simulink model "MIMO_code_pll_v2_r2016b"  (R2016b)
settings: Solver=FixedStepDiscrete  StartTime=0.0  StopTime=30  FixedStep=Ts  RelTol=1e-3
InitFcn:
  | Ts = 50e-6;
libraries: powerlib x16, powerlib_meascontrol x4
settings Model: Creator=ym  LastModifiedBy=ncepri14

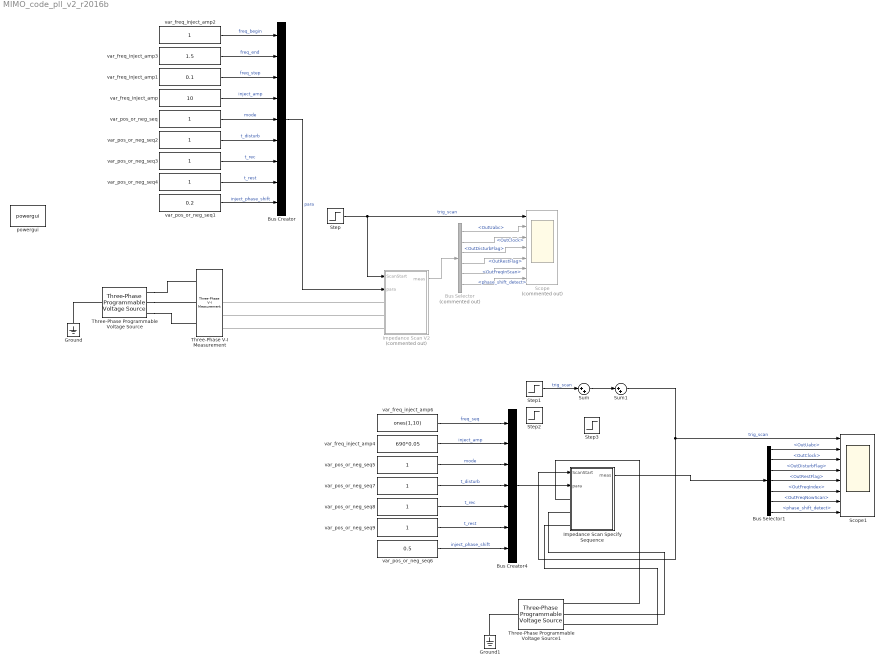
== system MIMO_code_pll_v2_r2016b ==
  Bus Creator : BusCreator  Inputs=9
  Bus Creator4 : BusCreator  Inputs=7
  Bus Selector : BusSelector  Commented=on  OutputSignals=scan_module_meas.OutUabc,scan_module_meas.OutClock,scan_module_meas.OutDisturbFlag,scan_module_meas.OutRestFlag,scan_module_meas.OutFreqInScan,phase_shift_detect
  Bus Selector1 : BusSelector  OutputSignals=scan_module_meas.OutUabc,scan_module_meas.OutClock,scan_module_meas.OutDisturbFlag,scan_module_meas.OutRestFlag,scan_module_meas.OutFreqIndex,scan_module_meas.OutFreqNowScan,phase_shift_detect
  Ground : powerlib/Elements/Ground  LConnTagsString=a
  Ground1 : powerlib/Elements/Ground  LConnTagsString=a
  Impedance Scan Specify Sequence : Subsystem  mask{var_gui_external=External, var_t_start=2, var_freq_seq=[1:350], var_inject_duration=1, var_record_duration=1, var_rest_duration=2, var_inject_amp=690*0.05, var_inject_mode=1, var_inject_phase_shift=0, var_ts=50e-6}
      mask prompts: var_gui_external "Using"; var_t_start "Injection starting time (s)"; var_freq_seq "Frequency Sequence (Hz)"; var_inject_duration "Injection durtion (s)"; var_record_duration "Record duration (s), this set only output a recording signal"; var_rest_duration "Stable durtion (s)"; var_inject_amp "Injection magnitude. eg. 690*0.02"; var_inject_mode "Injection mode. eg 1 for Positive sequence, 2 for Negative, 3 for MIMO"; var_inject_phase_shift "Injection phase shift angle (deg). eg. if set 20 deg, disturb will injected when the phase angle 20deg of grid Uabc comes"; var_ts "Sample time"
      mask help:
      | |--------------Injection duration--------------|-----Stable duration------|
      |                      |-----Record duration-----|
      |
      | Record duration <= Inject duration
      |
      | Freq coupling implemented in this version
      mask init:
      | block = find_system(gcb,...
      |           'LookUnderMasks','on',...
      |           'FollowLinks','on','Name','In2');
      | % p=Simulink.Mask.get(gcb);
      | 
      | maskObj = Simulink.Mask.get(gcb);
      | [control, phandle] = maskObj.getDialogControl('para_group_gui_setting_zone');
      | 
      | switch var_gui_external
      |     case 1
      |         
      | %       if ~isempty(block)
      | % %         delete_block(block);
      | %         
      | %       end
      |       control.Visible = 'on';
      | 
      |       
      |       
      | %       p.getDialogControl('para_group_gui_setting_zone').Visible='on';
      |     case 2
      |         
      | %         if isempty(block)
      | % %             add_block('built-in/Inport',[gcb,'/In2']);
      | %         end
      |         
      |         control.Visible = 'off';
      | %         p.getDialogControl('para_group_gui_setting_zone').Visible='off';
      | end % switch
      | 
      | disp(num2str(var_gui_external));
      mask Help:
      | by Yamin
      | v2(2024/5/17):
      | 1. add PLL phase alignment;
      | 2. Frequence sequence now can be specified by vector, elements could be random if you intend to do so.
      mask TypeOptions var_gui_external: GUI | External
  Impedance Scan V2 : Subsystem  Commented=on  mask{var_gui_external=External, t_start=2, freq_begin=1, freq_end=10, freq_step=1, inject_duration=1, record_duration=1, stable_duration=2, amp_inject=1, inject_mode=1, inject_phase_shift=30, var_ts=50e-6}
      mask prompts: var_gui_external "Using"; t_start "Injection starting time (s)"; freq_begin "Frequency begin (Hz)"; freq_end "Frequncy end (Hz)"; freq_step "Frequency step (Hz)"; inject_duration "Injection durtion (s)"; record_duration "Record duration (s), this set only output a recording signal"; stable_duration "Stable durtion (s)"; amp_inject "Injection magnitude. eg. 690*0.02"; inject_mode "Injection mode. eg 1 for Positive sequence, 2 for Negative, 3 for MIMO"; inject_phase_shift "Injection phase shift angle (deg). eg. if set 20 deg, disturb will injected when the phase angle 20deg of grid Uabc comes"; var_ts "Sample time"
      mask help:
      | |--------------Injection duration--------------|-----Stable duration------|
      |                      |-----Record duration-----|
      |
      | Record duration <= Inject duration
      |
      | Freq coupling implemented in this version
      mask init: same as MIMO_code_pll_v2_r2016b/Impedance Scan Specify Sequence
      mask Help: by Yamin
      mask TypeOptions var_gui_external: GUI | External
  Scope : Scope  Commented=on  NumInputPorts=7
  Scope1 : Scope  NumInputPorts=8
  Step : Step  SampleTime=0
  Step1 : Step  SampleTime=0
  Step2 : Step  Time=2  After=-1  SampleTime=0
  Step3 : Step  Time=5  SampleTime=0
  Sum : Sum  Inputs=|++
  Sum1 : Sum  Inputs=|++
  Three-Phase Programmable Voltage Source : powerlib/Electrical Sources/Three-Phase Programmable Voltage Source  PositiveSequence="[100  0 60]"  VariationEntity=None  VariationType=Table of time-amplitude pairs  VariationTypeAlt=Step  VariationStep=0.5  VariationRate=10  VariationMagnitude=0.3  VariationFrequency=2  VariationTiming=[1 2]  VariationPhaseA=off  Amplitudes=[1 0.8 1.2 1.0]  TimeValues=[0 0.1 0.15 0.2]  HarmonicGeneration=off  HarmonicA=[3 0.2 -25 0]  HarmonicB=[2 0.15 35 2]  Timing="[0.05  3]"  BusType=swing  Pref=0  Qref=0  Qmin=-inf  Qmax=inf
  Three-Phase Programmable Voltage Source1 : powerlib/Electrical Sources/Three-Phase Programmable Voltage Source  PositiveSequence="[100  0 60]"  VariationEntity=None  VariationType=Table of time-amplitude pairs  VariationTypeAlt=Step  VariationStep=0.5  VariationRate=10  VariationMagnitude=0.3  VariationFrequency=2  VariationTiming=[1 2]  VariationPhaseA=off  Amplitudes=[1 0.8 1.2 1.0]  TimeValues=[0 0.1 0.15 0.2]  HarmonicGeneration=off  HarmonicA=[3 0.2 -25 0]  HarmonicB=[2 0.15 35 2]  Timing="[0.05  3]"  BusType=swing  Pref=0  Qref=0  Qmin=-inf  Qmax=inf
  Three-Phase V-I Measurement : powerlib/Measurements/Three-Phase V-I Measurement  VoltageMeasurement=phase-to-ground  SetLabelV=off  LabelV=Vabc  Vpu=off  VpuLL=off  CurrentMeasurement=yes  SetLabelI=off  LabelI=Iabc  Ipu=off  Pbase=100e6  Vbase=500e3  OutputType=Complex  PhasorSimulation=off  PSBequivalent=0
  powergui : powerlib/powergui  Priority=1  SimulationMode=Discrete  SolverType=Tustin/Backward Euler (TBE)  SampleTime=Ts  frequency=60  SPID=off  DisableSnubberDevices=off  DisableRonSwitches=off  DisableVfSwitches=off  SwTol=0  DisplayEquations=off  Interpol=off  ExternalGateDelay=off  methode=off  Ts=10  FunctionMessages=off  echomessages=off  HookPort=off  EnableUseOfTLC=off  x0status=blocks  frequencyindice=60  Pbase=100e6  ErrMax=1e-4  Iterations=50  UnitsV=kV  UnitsW=MW  buscounter=0  RestoreLinks=warning  ResistiveCurrentMeasurement=off  Frange=[0:2:500]  Ylog=off  Xlog=on  ShowGrid=off  save=off  variable=ZData  structure=0  ZoomFFT=off  StartTime=0.0  cycles=1  DisplayStyle=1  fundamental=60  FreqAxis=off  MaxFrequency=1000  frequencyindicesteady=1  RmsSteady=1  display=off
  var_freq_inject_amp : Constant  Value=10
  var_freq_inject_amp1 : Constant  Value=0.1
  var_freq_inject_amp2 : Constant
  var_freq_inject_amp3 : Constant  Value=1.5
  var_freq_inject_amp4 : Constant  Value=690*0.05
  var_freq_inject_amp6 : Constant  Value=ones(1,10)
  var_pos_or_neg_seq{,2..5,7..9} (8 alike) : Constant
  var_pos_or_neg_seq1 : Constant  Value=0.2
  var_pos_or_neg_seq6 : Constant  Value=0.5
  wires:
  Impedance Scan V2/1(meas) -> Bus Selector/1
  var_freq_inject_amp1/1 -> Bus Creator/3  "freq_step"
  var_freq_inject_amp/1 -> Bus Creator/4  "inject_amp"
  var_pos_or_neg_seq/1 -> Bus Creator/5  "mode"
  var_pos_or_neg_seq2/1 -> Bus Creator/6  "t_disturb"
  var_pos_or_neg_seq3/1 -> Bus Creator/7  "t_rec"
  var_pos_or_neg_seq4/1 -> Bus Creator/8  "t_rest"
  var_freq_inject_amp2/1 -> Bus Creator/1  "freq_begin"
  var_freq_inject_amp3/1 -> Bus Creator/2  "freq_end"
  Step/1 -> Impedance Scan V2/1(ScanStart), Scope/1  "trig_scan"
  Bus Creator/1 -> Impedance Scan V2/2(para)  "para"
  var_pos_or_neg_seq1/1 -> Bus Creator/9  "inject_phase_shift"
  Bus Selector/3 -> Scope/4  "<OutDisturbFlag>"
  Bus Selector/2 -> Scope/3  "<OutClock>"
  Bus Selector/4 -> Scope/5  "<OutRestFlag>"
  Bus Selector/1 -> Scope/2  "<OutUabc>"
  Bus Selector/5 -> Scope/6  "<OutFreqInScan>"
  Bus Selector/6 -> Scope/7  "<phase_shift_detect>"
  var_freq_inject_amp4/1 -> Bus Creator4/2  "inject_amp"
  var_pos_or_neg_seq5/1 -> Bus Creator4/3  "mode"
  var_pos_or_neg_seq7/1 -> Bus Creator4/4  "t_disturb"
  var_pos_or_neg_seq8/1 -> Bus Creator4/5  "t_rec"
  var_pos_or_neg_seq9/1 -> Bus Creator4/6  "t_rest"
  var_freq_inject_amp6/1 -> Bus Creator4/1  "freq_seq"
  var_pos_or_neg_seq6/1 -> Bus Creator4/7  "inject_phase_shift"
  Bus Creator4/1 -> Impedance Scan Specify Sequence/2(para)
  Impedance Scan Specify Sequence/1(meas) -> Bus Selector1/1
  Sum1/1 -> Impedance Scan Specify Sequence/1(ScanStart), Scope1/1  "trig_scan"
  Step1/1 -> Sum/1  "trig_scan"
  Sum/1 -> Sum1/1
  Bus Selector1/4 -> Scope1/5  "<OutRestFlag>"
  Bus Selector1/3 -> Scope1/4  "<OutDisturbFlag>"
  Bus Selector1/5 -> Scope1/6  "<OutFreqIndex>"
  Bus Selector1/2 -> Scope1/3  "<OutClock>"
  Bus Selector1/6 -> Scope1/7  "<OutFreqNowScan>"
  Bus Selector1/1 -> Scope1/2  "<OutUabc>"
  Bus Selector1/7 -> Scope1/8  "<phase_shift_detect>"
  connections:
  Three-Phase Programmable Voltage Source/RConn3 -- Three-Phase V-I Measurement/LConn3
  Three-Phase Programmable Voltage Source/RConn2 -- Three-Phase V-I Measurement/LConn2
  Three-Phase Programmable Voltage Source/RConn1 -- Three-Phase V-I Measurement/LConn1
  Impedance Scan V2/LConn3 -- Three-Phase V-I Measurement/RConn3
  Impedance Scan V2/LConn2 -- Three-Phase V-I Measurement/RConn2
  Impedance Scan V2/LConn1 -- Three-Phase V-I Measurement/RConn1
  Ground/LConn1 -- Three-Phase Programmable Voltage Source/LConn1
  Ground1/LConn1 -- Three-Phase Programmable Voltage Source1/LConn1
  Impedance Scan Specify Sequence/LConn1 -- Three-Phase Programmable Voltage Source1/RConn1
  Impedance Scan Specify Sequence/LConn3 -- Three-Phase Programmable Voltage Source1/RConn3
  Impedance Scan Specify Sequence/LConn2 -- Three-Phase Programmable Voltage Source1/RConn2

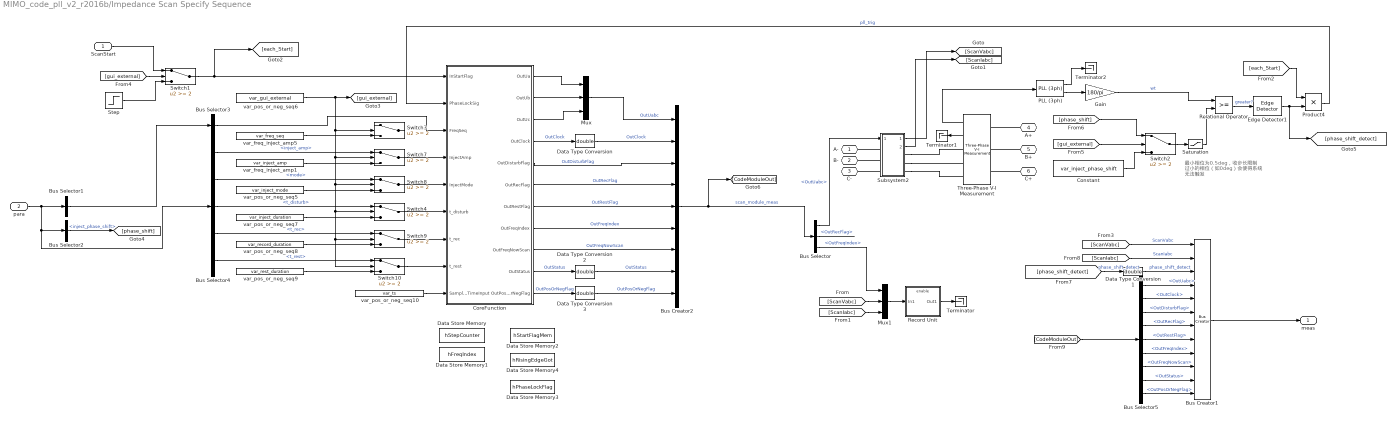
== system MIMO_code_pll_v2_r2016b/Impedance Scan Specify Sequence ==
  note: 最小相位为0.5deg，收步长限制
      | 过小的相位（如0deg）会使得系统
      | 无法触发
  ScanStart : Inport
  para : Inport  Port=2
  Bus Creator1 : BusCreator  Inputs=12
  Bus Creator2 : BusCreator  Inputs=9
  Bus Selector : BusSelector  OutputSignals=OutUabc,OutRecFlag,OutFreqIndex
  Bus Selector1 : BusSelector  OutputSignals=freq_seq,inject_amp,mode,t_disturb,t_rec,t_rest  OutputAsBus=on
  Bus Selector2 : BusSelector  OutputSignals=inject_phase_shift
  Bus Selector3 : BusSelector  OutputSignals=freq_seq  OutputAsBus=on
  Bus Selector4 : BusSelector  OutputSignals=inject_amp,mode,t_disturb,t_rec,t_rest
  Bus Selector5 : BusSelector  OutputSignals=OutUabc,OutClock,OutDisturbFlag,OutRecFlag,OutRestFlag,OutFreqIndex,OutFreqNowScan,OutStatus,OutPosOrNegFlag
  Constant : Constant  Value=var_inject_phase_shift
  CoreFunction : MATLAB Function  TreatAsAtomicUnit=on  SystemSampleTime=var_ts
  Data Store Memory : DataStoreMemory  DataStoreName=hStepCounter  ReadBeforeWriteMsg=warning  WriteAfterWriteMsg=warning  WriteAfterReadMsg=warning  ShowAdditionalParam=off  OutDataTypeStr=int32
  Data Store Memory1 : DataStoreMemory  DataStoreName=hFreqIndex  ReadBeforeWriteMsg=warning  WriteAfterWriteMsg=warning  WriteAfterReadMsg=warning  ShowAdditionalParam=off  OutDataTypeStr=double
  Data Store Memory2 : DataStoreMemory  DataStoreName=hStartFlagMem  ReadBeforeWriteMsg=warning  WriteAfterWriteMsg=warning  WriteAfterReadMsg=warning  ShowAdditionalParam=off  OutDataTypeStr=int32
  Data Store Memory3 : DataStoreMemory  DataStoreName=hPhaseLockFlag  ReadBeforeWriteMsg=warning  WriteAfterWriteMsg=warning  WriteAfterReadMsg=warning  ShowAdditionalParam=off  OutDataTypeStr=double
  Data Store Memory4 : DataStoreMemory  DataStoreName=hRisingEdgeGot  ReadBeforeWriteMsg=warning  WriteAfterWriteMsg=warning  WriteAfterReadMsg=warning  ShowAdditionalParam=off  OutDataTypeStr=double
  Data Type Conversion{,1..3} (4 alike) : DataTypeConversion  OutDataTypeStr=double
  Edge Detector1 : powerlib_meascontrol/Logic/Edge Detector  model=Rising  ic=0  Ts=var_ts
  Gain : Gain  Gain=180/pi
  Mux : Mux  Inputs=3
  Mux1 : Mux  Inputs=3
  PLL (3ph) : powerlib_meascontrol/PLL/PLL (3ph)  Fmin=45  Par_Init=[0, 50]  ParK=[180, 3200, 1]  TcD=1e-4  MaxRateChangeFreq=12  FilterCutOffFreq=25  Ts=var_ts  AGC=on
  Product4 : Product
  Record Unit : Subsystem
  Relational Operator : RelationalOperator  OutDataTypeStr=boolean  RndMeth=Simplest
  Saturation : Saturate  UpperLimit=inf  LowerLimit=0.5
  Step : Step  Time=var_t_start  SampleTime=0
  Subsystem2 : Subsystem
  Switch{1..2,4,7..10} (7 alike) : Switch  Threshold=2
  Switch3 : Switch  Threshold=2  AllowDiffInputSizes=on
  Terminator : Terminator
  Terminator1 : Terminator
  Terminator2 : Terminator
  Three-Phase V-I Measurement : powerlib/Measurements/Three-Phase V-I Measurement  VoltageMeasurement=phase-to-ground  SetLabelV=off  LabelV=Vabc  Vpu=off  VpuLL=off  CurrentMeasurement=yes  SetLabelI=off  LabelI=Iabc  Ipu=off  Pbase=100e6  Vbase=500e3  OutputType=Complex  PhasorSimulation=off  PSBequivalent=0
  var_freq_inject_amp1 : Constant  Value=var_inject_amp
  var_freq_inject_amp5 : Constant  Value=var_freq_seq
  var_pos_or_neg_seq10 : Constant  Value=var_ts
  var_pos_or_neg_seq5 : Constant  Value=var_inject_mode
  var_pos_or_neg_seq6 : Constant  Value=var_gui_external
  var_pos_or_neg_seq7 : Constant  Value=var_inject_duration
  var_pos_or_neg_seq8 : Constant  Value=var_record_duration
  var_pos_or_neg_seq9 : Constant  Value=var_rest_duration
  A- : PMIOPort  Port=1  Side=Left
  B- : PMIOPort  Port=2  Side=Left
  C- : PMIOPort  Port=3  Side=Left
  A+ : PMIOPort  Port=4  Side=Right
  B+ : PMIOPort  Port=5  Side=Right
  C+ : PMIOPort  Port=6  Side=Right
  meas : Outport
  wires:
  CoreFunction/9(OutFreqNowScan) -> Bus Creator2/7  "OutFreqNowScan"
  Bus Selector/2 -> ?  "<OutRecFlag>"
  Bus Selector1/1 -> Bus Selector3/1
  var_pos_or_neg_seq10/1 -> CoreFunction/9(SampleTimeInput)
  var_pos_or_neg_seq6/1 -> Switch3/2, Switch7/2, Switch8/2, Switch4/2, Switch9/2, Switch10/2, [gui_external]
  CoreFunction/8(OutFreqIndex) -> Bus Creator2/6  "OutFreqIndex"
  CoreFunction/7(OutRestFlag) -> Bus Creator2/5  "OutRestFlag"
  CoreFunction/5(OutDisturbFlag) -> Bus Creator2/3  "OutDisturbFlag"
  CoreFunction/6(OutRecFlag) -> Bus Creator2/4  "OutRecFlag"
  Data Type Conversion2/1 -> Bus Creator2/8  "OutStatus"
  Data Type Conversion/1 -> Bus Creator2/2  "OutClock"
  Data Type Conversion3/1 -> Bus Creator2/9  "OutPosOrNegFlag"
  Mux/1 -> Bus Creator2/1  "OutUabc"
  CoreFunction/1(OutUa) -> Mux/1
  CoreFunction/3(OutUc) -> Mux/3
  CoreFunction/2(OutUb) -> Mux/2
  Switch7/1 -> CoreFunction/4(InjectAmp)
  Switch8/1 -> CoreFunction/5(InjectMode)
  Switch4/1 -> CoreFunction/6(t_disturb)
  Switch9/1 -> CoreFunction/7(t_rec)
  Switch10/1 -> CoreFunction/8(t_rest)
  var_pos_or_neg_seq9/1 -> Switch10/3
  var_pos_or_neg_seq8/1 -> Switch9/3
  var_pos_or_neg_seq7/1 -> Switch4/3
  var_pos_or_neg_seq5/1 -> Switch8/3
  var_freq_inject_amp1/1 -> Switch7/3
  var_freq_inject_amp5/1 -> Switch3/3
  Bus Selector4/1 -> Switch7/1  "<inject_amp>"
  Bus Selector4/4 -> Switch9/1  "<t_rec>"
  Bus Selector4/3 -> Switch4/1  "<t_disturb>"
  Bus Selector4/5 -> Switch10/1  "<t_rest>"
  Bus Selector4/2 -> Switch8/1  "<mode>"
  Bus Selector3/1 -> CoreFunction/3(FreqSeq)
  CoreFunction/11(OutPosOrNegFlag) -> Data Type Conversion3/1  "OutPosOrNegFlag"
  CoreFunction/10(OutStatus) -> Data Type Conversion2/1  "OutStatus"
  CoreFunction/4(OutClock) -> Data Type Conversion/1  "OutClock"
  Subsystem2/2(Iabc) -> [ScanIabc]
  Subsystem2/1(Uabc) -> [ScanVabc]
  Bus Selector/3 -> Mux1/1  "<OutFreqIndex>"
  Mux1/1 -> Record Unit/1(In1)
  Record Unit/1(Out1) -> Terminator/1
  [ScanIabc] -> Mux1/3
  [ScanVabc] -> Mux1/2
  Bus Selector/1 -> Subsystem2/1(In1)  "<OutUabc>"
  Bus Creator2/1 -> [CodeModuleOut], Bus Selector/1  "scan_module_meas"
  Three-Phase V-I Measurement/1 -> PLL (3ph)/1
  PLL (3ph)/2 -> Gain/1
  Gain/1 -> Relational Operator/1  "wt"
  Constant/1 -> Switch2/3
  Relational Operator/1 -> Edge Detector1/1  "greater?"
  Product4/1 -> CoreFunction/2(PhaseLockSig)  "pll_trig"
  [each_Start] -> Product4/1
  Switch1/1 -> [each_Start], CoreFunction/1(InStartFlag)
  ScanStart/1 -> Switch1/1
  Step/1 -> Switch1/3
  Three-Phase V-I Measurement/2 -> Terminator1/1
  Saturation/1 -> Relational Operator/2
  [gui_external] -> Switch2/2
  [gui_external] -> Switch1/2
  para/1 -> Bus Selector1/1, Bus Selector4/1, Bus Selector2/1
  Bus Selector2/1 -> [phase_shift]  "<inject_phase_shift>"
  [phase_shift] -> Switch2/1
  Bus Creator1/1 -> meas/1
  PLL (3ph)/1 -> Terminator2/1
  [phase_shift_detect] -> Data Type Conversion1/1  "phase_shift_detect"
  Edge Detector1/1 -> [phase_shift_detect], Product4/2
  Switch2/1 -> Saturation/1
  Data Type Conversion1/1 -> Bus Creator1/3  "phase_shift_detect"
  [ScanVabc] -> Bus Creator1/1  "ScanVabc"
  [ScanIabc] -> Bus Creator1/2  "ScanIabc"
  Bus Selector5/3 -> Bus Creator1/6  "<OutDisturbFlag>"
  Bus Selector5/2 -> Bus Creator1/5  "<OutClock>"
  Bus Selector5/4 -> Bus Creator1/7  "<OutRecFlag>"
  Bus Selector5/1 -> Bus Creator1/4  "<OutUabc>"
  Bus Selector5/5 -> Bus Creator1/8  "<OutRestFlag>"
  Bus Selector5/6 -> Bus Creator1/9  "<OutFreqIndex>"
  Bus Selector5/7 -> Bus Creator1/10  "<OutFreqNowScan>"
  Bus Selector5/8 -> Bus Creator1/11  "<OutStatus>"
  Bus Selector5/9 -> Bus Creator1/12  "<OutPosOrNegFlag>"
  [CodeModuleOut] -> Bus Selector5/1
  connections:
  Subsystem2/LConn3 -- C-/RConn1
  Subsystem2/LConn2 -- B-/RConn1
  Subsystem2/LConn1 -- A-/RConn1
  B+/RConn1 -- Three-Phase V-I Measurement/LConn2
  C+/RConn1 -- Three-Phase V-I Measurement/LConn3
  A+/RConn1 -- Three-Phase V-I Measurement/LConn1
  Subsystem2/RConn1 -- Three-Phase V-I Measurement/RConn1
  Subsystem2/RConn2 -- Three-Phase V-I Measurement/RConn2
  Subsystem2/RConn3 -- Three-Phase V-I Measurement/RConn3

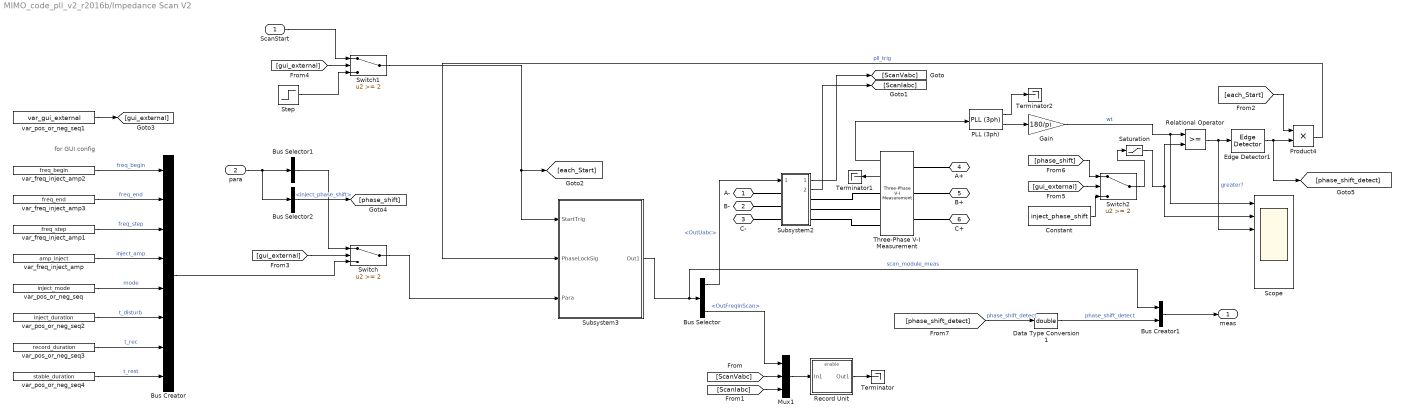
== system MIMO_code_pll_v2_r2016b/Impedance Scan V2 ==
  note: for GUI config
  ScanStart : Inport
  para : Inport  Port=2
  Bus Creator : BusCreator  Inputs=8
  Bus Creator1 : BusCreator  Inputs=2
  Bus Selector : BusSelector  OutputSignals=OutUabc,OutRecFlag,OutFreqInScan
  Bus Selector1 : BusSelector  OutputSignals=freq_begin,freq_end,freq_step,inject_amp,mode,t_disturb,t_rec,t_rest  OutputAsBus=on
  Bus Selector2 : BusSelector  OutputSignals=inject_phase_shift
  Constant : Constant  Value=inject_phase_shift
  Data Type Conversion1 : DataTypeConversion  OutDataTypeStr=double
  Edge Detector1 : powerlib_meascontrol/Logic/Edge Detector  model=Rising  ic=0  Ts=var_ts
  Gain : Gain  Gain=180/pi
  Mux1 : Mux  Inputs=3
  PLL (3ph) : powerlib_meascontrol/PLL/PLL (3ph)  Fmin=45  Par_Init=[0, 50]  ParK=[180, 3200, 1]  TcD=1e-4  MaxRateChangeFreq=12  FilterCutOffFreq=25  Ts=var_ts  AGC=on
  Product4 : Product
  Record Unit : Subsystem
  Relational Operator : RelationalOperator  OutDataTypeStr=boolean  RndMeth=Simplest
  Saturation : Saturate  UpperLimit=inf  LowerLimit=0.5
  Scope : Scope  NumInputPorts=7
  Step : Step  Time=t_start  SampleTime=0
  Subsystem2 : Subsystem
  Subsystem3 : Subsystem  mask{var_gui_external=External, var_freq_begin=1, var_freq_end=1, var_freq_step=1, var_freq_inject_amp=amp_inject, var_t_disturb=inject_duration, var_t_rec=record_duration, var_t_rest=stable_duration, var_inject_mode=inject_mode}
      mask prompts: var_gui_external "Set Parameters using GUI or External"; var_freq_begin "FreqBegin"; var_freq_end "FreqEnd"; var_freq_step "FreqStep"; var_freq_inject_amp "FreqInjectAmp"; var_t_disturb "T disturbance"; var_t_rec "T recording"; var_t_rest "T rest"; var_inject_mode "Positve or Negative Sequence"
      mask init: same as MIMO_code_pll_v2_r2016b/Impedance Scan Specify Sequence
      mask TypeOptions var_gui_external: GUI | External
      mask DialogControl para_group_gui_setting_zone Prompt: GUI Setting Zone
  Switch : Switch  Threshold=2
  Switch1 : Switch  Threshold=2
  Switch2 : Switch  Threshold=2
  Terminator : Terminator
  Terminator1 : Terminator
  Terminator2 : Terminator
  Three-Phase V-I Measurement : powerlib/Measurements/Three-Phase V-I Measurement  VoltageMeasurement=phase-to-ground  SetLabelV=off  LabelV=Vabc  Vpu=off  VpuLL=off  CurrentMeasurement=yes  SetLabelI=off  LabelI=Iabc  Ipu=off  Pbase=100e6  Vbase=500e3  OutputType=Complex  PhasorSimulation=off  PSBequivalent=0
  var_freq_inject_amp : Constant  Value=amp_inject
  var_freq_inject_amp1 : Constant  Value=freq_step
  var_freq_inject_amp2 : Constant  Value=freq_begin
  var_freq_inject_amp3 : Constant  Value=freq_end
  var_pos_or_neg_seq : Constant  Value=inject_mode
  var_pos_or_neg_seq1 : Constant  Value=var_gui_external
  var_pos_or_neg_seq2 : Constant  Value=inject_duration
  var_pos_or_neg_seq3 : Constant  Value=record_duration
  var_pos_or_neg_seq4 : Constant  Value=stable_duration
  A- : PMIOPort  Port=1  Side=Left
  B- : PMIOPort  Port=2  Side=Left
  C- : PMIOPort  Port=3  Side=Left
  A+ : PMIOPort  Port=4  Side=Right
  B+ : PMIOPort  Port=5  Side=Right
  C+ : PMIOPort  Port=6  Side=Right
  meas : Outport
  wires:
  Subsystem2/2(Iabc) -> [ScanIabc]
  Subsystem2/1(Uabc) -> [ScanVabc]
  Bus Selector/3 -> Mux1/1  "<OutFreqInScan>"
  Mux1/1 -> Record Unit/1(In1)
  Record Unit/1(Out1) -> Terminator/1
  [ScanIabc] -> Mux1/3
  [ScanVabc] -> Mux1/2
  Bus Selector/1 -> Subsystem2/1(In1)  "<OutUabc>"
  Subsystem3/1(Out1) -> Bus Creator1/1, Bus Selector/1  "scan_module_meas"
  Three-Phase V-I Measurement/1 -> PLL (3ph)/1
  PLL (3ph)/2 -> Gain/1
  Gain/1 -> Relational Operator/1, Scope/1  "wt"
  Constant/1 -> Switch2/3
  Relational Operator/1 -> Scope/3, Edge Detector1/1  "greater?"
  Product4/1 -> Subsystem3/2(PhaseLockSig)  "pll_trig"
  [each_Start] -> Product4/1
  Switch1/1 -> Subsystem3/1(StartTrig), [each_Start]
  var_freq_inject_amp1/1 -> Bus Creator/3  "freq_step"
  var_freq_inject_amp/1 -> Bus Creator/4  "inject_amp"
  var_pos_or_neg_seq/1 -> Bus Creator/5  "mode"
  var_pos_or_neg_seq2/1 -> Bus Creator/6  "t_disturb"
  var_pos_or_neg_seq3/1 -> Bus Creator/7  "t_rec"
  var_pos_or_neg_seq4/1 -> Bus Creator/8  "t_rest"
  var_freq_inject_amp2/1 -> Bus Creator/1  "freq_begin"
  var_freq_inject_amp3/1 -> Bus Creator/2  "freq_end"
  [gui_external] -> Switch/2
  Bus Creator/1 -> Switch/3
  Switch/1 -> Subsystem3/3(Para)
  ScanStart/1 -> Switch1/1
  Step/1 -> Switch1/3
  Three-Phase V-I Measurement/2 -> Terminator1/1
  Saturation/1 -> Relational Operator/2, Scope/2
  [gui_external] -> Switch2/2
  var_pos_or_neg_seq1/1 -> [gui_external]
  [gui_external] -> Switch1/2
  para/1 -> Bus Selector2/1, Bus Selector1/1
  Bus Selector2/1 -> [phase_shift]  "<inject_phase_shift>"
  [phase_shift] -> Switch2/1
  Bus Creator1/1 -> meas/1
  PLL (3ph)/1 -> Terminator2/1
  [phase_shift_detect] -> Data Type Conversion1/1  "phase_shift_detect"
  Edge Detector1/1 -> [phase_shift_detect], Product4/2
  Bus Selector1/1 -> Switch/1
  Switch2/1 -> Saturation/1
  Data Type Conversion1/1 -> Bus Creator1/2  "phase_shift_detect"
  connections:
  Subsystem2/LConn3 -- C-/RConn1
  Subsystem2/LConn2 -- B-/RConn1
  Subsystem2/LConn1 -- A-/RConn1
  B+/RConn1 -- Three-Phase V-I Measurement/LConn2
  C+/RConn1 -- Three-Phase V-I Measurement/LConn3
  A+/RConn1 -- Three-Phase V-I Measurement/LConn1
  Subsystem2/RConn1 -- Three-Phase V-I Measurement/RConn1
  Subsystem2/RConn2 -- Three-Phase V-I Measurement/RConn2
  Subsystem2/RConn3 -- Three-Phase V-I Measurement/RConn3

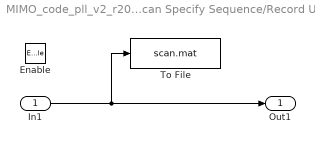
== system MIMO_code_pll_v2_r2016b/Impedance Scan Specify Sequence/Record Unit ==
  In1 : Inport
  Enable : EnablePort
  To File : ToFile  Filename=scan.mat  MatrixName=scan  SampleTime=var_ts
  Out1 : Outport
  wires:
  In1/1 -> Out1/1, To File/1

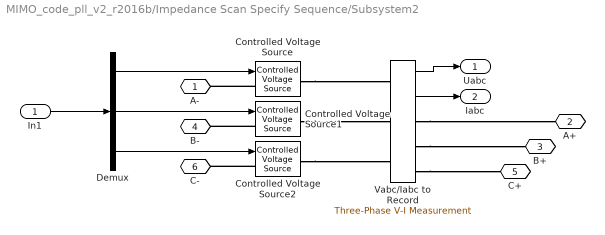
== system MIMO_code_pll_v2_r2016b/Impedance Scan Specify Sequence/Subsystem2 ==
  In1 : Inport
  Controlled Voltage Source : powerlib/Electrical Sources/Controlled Voltage Source  Initialize=on  Source_Type=AC  Amplitude=0  Phase=0  Frequency=0  Measurements=None
  Controlled Voltage Source1 : powerlib/Electrical Sources/Controlled Voltage Source  Initialize=on  Source_Type=AC  Amplitude=0  Phase=0  Frequency=0  Measurements=None
  Controlled Voltage Source2 : powerlib/Electrical Sources/Controlled Voltage Source  Initialize=on  Source_Type=AC  Amplitude=0  Phase=0  Frequency=0  Measurements=None
  Demux : Demux  Outputs=3
  Vabc/Iabc to Record : powerlib/Measurements/Three-Phase V-I Measurement  VoltageMeasurement=phase-to-ground  SetLabelV=off  LabelV=ScanVabc  Vpu=off  VpuLL=off  CurrentMeasurement=yes  SetLabelI=off  LabelI=ScanIabc  Ipu=off  Pbase=100e6  Vbase=500e3  OutputType=Complex  PhasorSimulation=off  PSBequivalent=0
  A- : PMIOPort  Port=1  Side=Left
  A+ : PMIOPort  Port=2  Side=Right
  B+ : PMIOPort  Port=3  Side=Right
  B- : PMIOPort  Port=4  Side=Left
  C+ : PMIOPort  Port=5  Side=Right
  C- : PMIOPort  Port=6  Side=Left
  Uabc : Outport
  Iabc : Outport  Port=2
  wires:
  Vabc/Iabc to Record/2 -> Iabc/1
  Vabc/Iabc to Record/1 -> Uabc/1
  In1/1 -> Demux/1
  Demux/1 -> Controlled Voltage Source/1
  Demux/2 -> Controlled Voltage Source1/1
  Demux/3 -> Controlled Voltage Source2/1
  connections:
  Controlled Voltage Source2/LConn1 -- C-/RConn1
  Vabc/Iabc to Record/RConn2 -- B+/RConn1
  Controlled Voltage Source1/LConn1 -- B-/RConn1
  Controlled Voltage Source/LConn1 -- A-/RConn1
  Vabc/Iabc to Record/RConn3 -- C+/RConn1
  Controlled Voltage Source2/RConn1 -- Vabc/Iabc to Record/LConn3
  Controlled Voltage Source1/RConn1 -- Vabc/Iabc to Record/LConn2
  Controlled Voltage Source/RConn1 -- Vabc/Iabc to Record/LConn1
  Vabc/Iabc to Record/RConn1 -- A+/RConn1

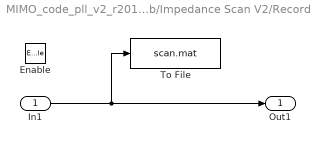
== system MIMO_code_pll_v2_r2016b/Impedance Scan V2/Record Unit ==
  In1 : Inport
  Enable : EnablePort
  To File : ToFile  Filename=scan.mat  MatrixName=scan  SampleTime=var_ts
  Out1 : Outport
  wires:
  In1/1 -> Out1/1, To File/1

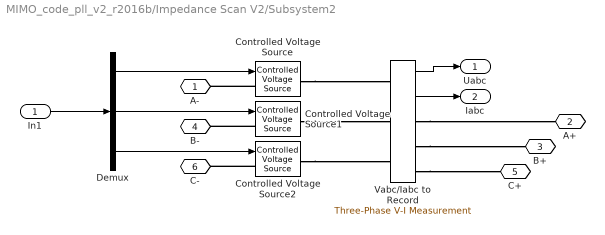
== system MIMO_code_pll_v2_r2016b/Impedance Scan V2/Subsystem2 ==
  In1 : Inport
  Controlled Voltage Source : powerlib/Electrical Sources/Controlled Voltage Source  Initialize=on  Source_Type=AC  Amplitude=0  Phase=0  Frequency=0  Measurements=None
  Controlled Voltage Source1 : powerlib/Electrical Sources/Controlled Voltage Source  Initialize=on  Source_Type=AC  Amplitude=0  Phase=0  Frequency=0  Measurements=None
  Controlled Voltage Source2 : powerlib/Electrical Sources/Controlled Voltage Source  Initialize=on  Source_Type=AC  Amplitude=0  Phase=0  Frequency=0  Measurements=None
  Demux : Demux  Outputs=3
  Vabc/Iabc to Record : powerlib/Measurements/Three-Phase V-I Measurement  VoltageMeasurement=phase-to-ground  SetLabelV=off  LabelV=ScanVabc  Vpu=off  VpuLL=off  CurrentMeasurement=yes  SetLabelI=off  LabelI=ScanIabc  Ipu=off  Pbase=100e6  Vbase=500e3  OutputType=Complex  PhasorSimulation=off  PSBequivalent=0
  A- : PMIOPort  Port=1  Side=Left
  A+ : PMIOPort  Port=2  Side=Right
  B+ : PMIOPort  Port=3  Side=Right
  B- : PMIOPort  Port=4  Side=Left
  C+ : PMIOPort  Port=5  Side=Right
  C- : PMIOPort  Port=6  Side=Left
  Uabc : Outport
  Iabc : Outport  Port=2
  wires:
  Vabc/Iabc to Record/2 -> Iabc/1
  Vabc/Iabc to Record/1 -> Uabc/1
  In1/1 -> Demux/1
  Demux/1 -> Controlled Voltage Source/1
  Demux/2 -> Controlled Voltage Source1/1
  Demux/3 -> Controlled Voltage Source2/1
  connections:
  Controlled Voltage Source2/LConn1 -- C-/RConn1
  Vabc/Iabc to Record/RConn2 -- B+/RConn1
  Controlled Voltage Source1/LConn1 -- B-/RConn1
  Controlled Voltage Source/LConn1 -- A-/RConn1
  Vabc/Iabc to Record/RConn3 -- C+/RConn1
  Controlled Voltage Source2/RConn1 -- Vabc/Iabc to Record/LConn3
  Controlled Voltage Source1/RConn1 -- Vabc/Iabc to Record/LConn2
  Controlled Voltage Source/RConn1 -- Vabc/Iabc to Record/LConn1
  Vabc/Iabc to Record/RConn1 -- A+/RConn1

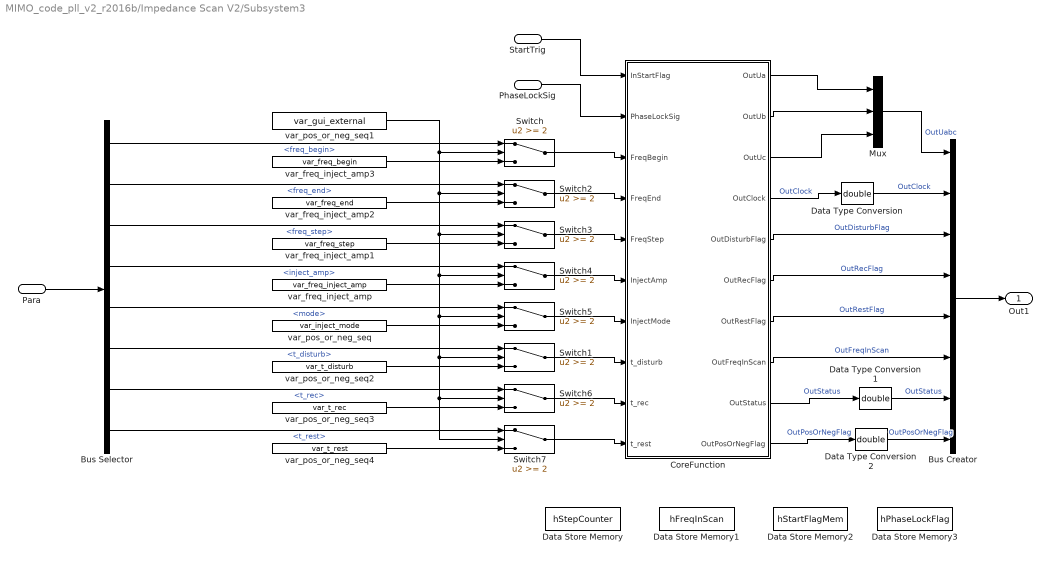
== system MIMO_code_pll_v2_r2016b/Impedance Scan V2/Subsystem3 ==
  StartTrig : Inport
  PhaseLockSig : Inport  Port=2
  Para : Inport  Port=3
  Bus Creator : BusCreator  Inputs=8
  Bus Selector : BusSelector  OutputSignals=freq_begin,freq_end,freq_step,inject_amp,mode,t_disturb,t_rec,t_rest
  CoreFunction : MATLAB Function  TreatAsAtomicUnit=on  SystemSampleTime=var_ts
  Data Store Memory : DataStoreMemory  DataStoreName=hStepCounter  ReadBeforeWriteMsg=warning  WriteAfterWriteMsg=warning  WriteAfterReadMsg=warning  ShowAdditionalParam=off  OutDataTypeStr=int32
  Data Store Memory1 : DataStoreMemory  DataStoreName=hFreqInScan  ReadBeforeWriteMsg=warning  WriteAfterWriteMsg=warning  WriteAfterReadMsg=warning  ShowAdditionalParam=off  OutDataTypeStr=double
  Data Store Memory2 : DataStoreMemory  DataStoreName=hStartFlagMem  ReadBeforeWriteMsg=warning  WriteAfterWriteMsg=warning  WriteAfterReadMsg=warning  ShowAdditionalParam=off  OutDataTypeStr=int32
  Data Store Memory3 : DataStoreMemory  DataStoreName=hPhaseLockFlag  ReadBeforeWriteMsg=warning  WriteAfterWriteMsg=warning  WriteAfterReadMsg=warning  ShowAdditionalParam=off  OutDataTypeStr=double
  Data Type Conversion : DataTypeConversion  OutDataTypeStr=double
  Data Type Conversion1 : DataTypeConversion  OutDataTypeStr=double
  Data Type Conversion2 : DataTypeConversion  OutDataTypeStr=double
  Mux : Mux  Inputs=3
  Switch{,1..7} (8 alike) : Switch  Threshold=2
  var_freq_inject_amp : Constant  Value=var_freq_inject_amp
  var_freq_inject_amp1 : Constant  Value=var_freq_step
  var_freq_inject_amp2 : Constant  Value=var_freq_end
  var_freq_inject_amp3 : Constant  Value=var_freq_begin
  var_pos_or_neg_seq : Constant  Value=var_inject_mode
  var_pos_or_neg_seq1 : Constant  Value=var_gui_external
  var_pos_or_neg_seq2 : Constant  Value=var_t_disturb
  var_pos_or_neg_seq3 : Constant  Value=var_t_rec
  var_pos_or_neg_seq4 : Constant  Value=var_t_rest
  Out1 : Outport
  wires:
  CoreFunction/8(OutFreqInScan) -> Bus Creator/6  "OutFreqInScan"
  CoreFunction/7(OutRestFlag) -> Bus Creator/5  "OutRestFlag"
  CoreFunction/5(OutDisturbFlag) -> Bus Creator/3  "OutDisturbFlag"
  CoreFunction/6(OutRecFlag) -> Bus Creator/4  "OutRecFlag"
  Data Type Conversion1/1 -> Bus Creator/7  "OutStatus"
  Data Type Conversion/1 -> Bus Creator/2  "OutClock"
  Bus Creator/1 -> Out1/1
  Data Type Conversion2/1 -> Bus Creator/8  "OutPosOrNegFlag"
  Mux/1 -> Bus Creator/1  "OutUabc"
  CoreFunction/1(OutUa) -> Mux/1
  CoreFunction/3(OutUc) -> Mux/3
  CoreFunction/2(OutUb) -> Mux/2
  Switch/1 -> CoreFunction/3(FreqBegin)
  Switch2/1 -> CoreFunction/4(FreqEnd)
  Switch3/1 -> CoreFunction/5(FreqStep)
  Switch4/1 -> CoreFunction/6(InjectAmp)
  Switch5/1 -> CoreFunction/7(InjectMode)
  Switch1/1 -> CoreFunction/8(t_disturb)
  Switch6/1 -> CoreFunction/9(t_rec)
  Switch7/1 -> CoreFunction/10(t_rest)
  var_pos_or_neg_seq1/1 -> Switch/2, Switch4/2, Switch7/2, Switch6/2, Switch1/2, Switch5/2, Switch3/2, Switch2/2
  StartTrig/1 -> CoreFunction/1(InStartFlag)
  var_pos_or_neg_seq4/1 -> Switch7/3
  var_pos_or_neg_seq3/1 -> Switch6/3
  var_pos_or_neg_seq2/1 -> Switch1/3
  var_pos_or_neg_seq/1 -> Switch5/3
  var_freq_inject_amp/1 -> Switch4/3
  var_freq_inject_amp1/1 -> Switch3/3
  var_freq_inject_amp2/1 -> Switch2/3
  var_freq_inject_amp3/1 -> Switch/3
  Bus Selector/4 -> Switch4/1  "<inject_amp>"
  Bus Selector/7 -> Switch6/1  "<t_rec>"
  Bus Selector/6 -> Switch1/1  "<t_disturb>"
  Bus Selector/8 -> Switch7/1  "<t_rest>"
  Bus Selector/5 -> Switch5/1  "<mode>"
  Bus Selector/3 -> Switch3/1  "<freq_step>"
  Bus Selector/2 -> Switch2/1  "<freq_end>"
  Bus Selector/1 -> Switch/1  "<freq_begin>"
  PhaseLockSig/1 -> CoreFunction/2(PhaseLockSig)
  Para/1 -> Bus Selector/1
  CoreFunction/10(OutPosOrNegFlag) -> Data Type Conversion2/1  "OutPosOrNegFlag"
  CoreFunction/9(OutStatus) -> Data Type Conversion1/1  "OutStatus"
  CoreFunction/4(OutClock) -> Data Type Conversion/1  "OutClock"

== matlab function MIMO_code_pll_v2_r2016b/Impedance Scan Specify Sequence/CoreFunction ==
  data: InStartFlag input; PhaseLockSig input; FreqSeq input; OutUa output; InjectAmp input; InjectMode input; t_disturb input; t_rec input; t_rest input; OutUb output; OutUc output; OutClock output; OutDisturbFlag output; OutRecFlag output; OutRestFlag output; OutFreqIndex output; OutFreqNowScan output; OutStatus output; OutPosOrNegFlag output; hStepCounter data_store_memory; hFreqIndex data_store_memory; hStartFlagMem data_store_memory; hPhaseLockFlag data_store_memory; SampleTimeInput input; hRisingEdgeGot data_store_memory
function [OutUa, OutUb, OutUc, ...
    OutClock, OutDisturbFlag, OutRecFlag, OutRestFlag, ...
    OutFreqIndex, OutFreqNowScan, OutStatus, OutPosOrNegFlag] = ...
    fcn(InStartFlag, PhaseLockSig, FreqSeq, InjectAmp, InjectMode, ...
    t_disturb, t_rec, t_rest, SampleTimeInput)
% InjectMode = 1, Positive sequence
% InjectMode = 2, Negative sequence
% InjectMode = 3, Positive et Negative simutaneously

global hStepCounter;
global hFreqIndex; 
global hStartFlagMem;
global hPhaseLockFlag;
global hRisingEdgeGot; % record a rising-edge get event, cleared untile all frequency are scanned.

this_freq = 0; %% only used for output
FreqSeqLength = length(FreqSeq);

SAMPLE_TIME = SampleTimeInput;
SAMPLE_FREQ = 1/SAMPLE_TIME;

T_DISTURB	= t_disturb * SAMPLE_FREQ;
T_REC 		= t_rec * SAMPLE_FREQ;
T_REST 		= t_rest * SAMPLE_FREQ;

clock_t		= 0;
start_flag	= 0;
status_code	= 0;
ua			= 0; 
ub			= 0; 
uc			= 0;
omega		= 0;
disturb_flag = 0;
rec_flag    = 0;
rest_flag   = 0;

if hPhaseLockFlag == 0 && PhaseLockSig == 1  % Phase-lock event catch, reset by every scan step
    hPhaseLockFlag = 1;
end


start_flag = InStartFlag;
if (start_flag >= 1 && hStartFlagMem == 0) % rising-edge event catch
	hRisingEdgeGot = 1;
	hFreqIndex = 1;
end

if (start_flag >= 1 && hRisingEdgeGot == 1) % once triggerd, loop untill all frequences are scanned
	if (hFreqIndex >=1 && hFreqIndex <= FreqSeqLength && hPhaseLockFlag == 1)
		status_code = 1;
		if (hStepCounter <= (T_DISTURB - T_REC))
			disturb_flag = 1;
			rec_flag = 0;
			rest_flag = 0;
			hStepCounter = hStepCounter + 1;
        elseif ((hStepCounter > (T_DISTURB - T_REC)) && (hStepCounter <= T_DISTURB) && hPhaseLockFlag == 1)
			disturb_flag = 1;
			rec_flag = 1;
			rest_flag = 0;
			hStepCounter = hStepCounter + 1;
        elseif ((hStepCounter > T_DISTURB) && hStepCounter <= (T_DISTURB + T_REST) && hPhaseLockFlag == 1)
			disturb_flag = 0;
			rec_flag = 0;
			rest_flag = 1;
			hStepCounter = hStepCounter + 1;
        else
			hStepCounter = int32(0);
			hFreqIndex = hFreqIndex + 1;
			ua = 0; ub = 0; uc = 0;
            hPhaseLockFlag = 0;
        end

		if (disturb_flag == 1) 
            this_freq = FreqSeq(hFreqIndex); % only used for output port 
			clock_t = double(hStepCounter) * SAMPLE_TIME;
			omega = 2.0 * FreqSeq(hFreqIndex) * pi;
            
			if (InjectMode == 1)
				ua = InjectAmp * sin(omega * clock_t);
				ub = InjectAmp * sin(omega * clock_t - 2.0*pi/3.0);
				uc = InjectAmp * sin(omega * clock_t + 2.0*pi/3.0);
			
            elseif (InjectMode == 2)
				ua = InjectAmp * sin(omega * clock_t);
				ub = InjectAmp * sin(omega * clock_t + 2.0*pi/3.0);
				uc = InjectAmp * sin(omega * clock_t - 2.0*pi/3.0);
                
            elseif (InjectMode == 3)
                ua = InjectAmp * sin(omega * clock_t);
				ub = 0.5 * InjectAmp * sin(omega * clock_t + 2.0*pi/3.0) + ...
                     0.5 * InjectAmp * sin(omega * clock_t - 2.0*pi/3.0);
				uc = ub;
            else
                % other InjectMode to be write here.
            end
        end
	elseif hFreqIndex > FreqSeqLength
		status_code = 2;
		hRisingEdgeGot = 0;
		ua = 0; ub = 0; uc = 0;
	else
		ua = 0; ub = 0; uc = 0;
		status_code = 3;
	end

else % start_flag == 0 || hRisingEdgeGot == 0

	hFreqIndex = 1;

	status_code = 0;
	disturb_flag = 0;
	rec_flag = 0;
	rest_flag = 0;
	hStepCounter = int32(0);
	clock_t = double(hStepCounter) * SAMPLE_TIME;
	ua = 0; ub = 0; uc = 0;
end
	hStartFlagMem = int32(start_flag);  % record start_flag
	OutUa = ua;
	OutUb = ub;
	OutUc = uc;

	OutStatus = status_code;
	OutFreqIndex = hFreqIndex;
	OutFreqNowScan = this_freq;
	OutClock = clock_t;
	OutDisturbFlag = disturb_flag;
	OutRecFlag = rec_flag;
	OutRestFlag = rest_flag;
    OutPosOrNegFlag = InjectMode;
end

== matlab function MIMO_code_pll_v2_r2016b/Impedance Scan V2/Subsystem3/CoreFunction ==
  data: InStartFlag input; PhaseLockSig input; FreqBegin input; OutUa output; FreqEnd input; FreqStep input; InjectAmp input; InjectMode input; t_disturb input; t_rec input; t_rest input; OutUb output; OutUc output; OutClock output; OutDisturbFlag output; OutRecFlag output; OutRestFlag output; OutFreqInScan output; OutStatus output; OutPosOrNegFlag output; hStepCounter data_store_memory; hFreqInScan data_store_memory; hStartFlagMem data_store_memory; hPhaseLockFlag data_store_memory
function [OutUa, OutUb, OutUc, ...
    OutClock, OutDisturbFlag, OutRecFlag, OutRestFlag, ...
    OutFreqInScan, OutStatus, OutPosOrNegFlag] = ...
    fcn(InStartFlag, PhaseLockSig, FreqBegin, FreqEnd, FreqStep, InjectAmp, InjectMode, ...
    t_disturb, t_rec, t_rest)
% InjectMode = 1, Positive sequence
% InjectMode = 2, Negative sequence
% InjectMode = 3, Positive et Negative simutaneously

global hStepCounter;
global hFreqInScan; 
global hStartFlagMem;
global hPhaseLockFlag;

SAMPLE_FREQ = 1/50e-6;
SAMPLE_TIME = 1/SAMPLE_FREQ;

T_DISTURB	= t_disturb * SAMPLE_FREQ;
T_REC 		= t_rec * SAMPLE_FREQ;
T_REST 		= t_rest * SAMPLE_FREQ;

clock_t		= 0;
start_flag	= 0;
status_code	= 0;
ua			= 0; 
ub			= 0; 
uc			= 0;
omega		= 0;
disturb_flag = 0;
rec_flag    = 0;
rest_flag   = 0;

if hPhaseLockFlag == 0 && PhaseLockSig == 1
    hPhaseLockFlag = 1;
end

start_flag = InStartFlag;
	if (start_flag >= 1 && hFreqInScan >= FreqBegin)
		if (hStartFlagMem == 0)
			hFreqInScan = FreqBegin;
			status_code = -1;
        end
		
		if ((hFreqInScan >= FreqBegin) && (hFreqInScan <= FreqEnd) && hPhaseLockFlag == 1)
			status_code = 1;
			if (hStepCounter <= (T_DISTURB - T_REC))
				disturb_flag = 1;
				rec_flag = 0;
				rest_flag = 0;
				hStepCounter = hStepCounter + 1;
            elseif ((hStepCounter > (T_DISTURB - T_REC)) && (hStepCounter <= T_DISTURB) && hPhaseLockFlag == 1)
				disturb_flag = 1;
				rec_flag = 1;
				rest_flag = 0;
				hStepCounter = hStepCounter + 1;
            elseif ((hStepCounter > T_DISTURB) && hStepCounter <= (T_DISTURB + T_REST) && hPhaseLockFlag == 1)
				disturb_flag = 0;
				rec_flag = 0;
				rest_flag = 1;
				hStepCounter = hStepCounter + 1;
            else
				hStepCounter = int32(0);
				hFreqInScan = hFreqInScan + FreqStep;
				ua = 0; ub = 0; uc = 0;
                hPhaseLockFlag = 0;
            end

			if (disturb_flag == 1) 
				clock_t = double(hStepCounter) * SAMPLE_TIME;
				omega = 2.0 * hFreqInScan * pi;
                
				if (InjectMode == 1)
					ua = InjectAmp * sin(omega * clock_t);
					ub = InjectAmp * sin(omega * clock_t - 2.0*pi/3.0);
					uc = InjectAmp * sin(omega * clock_t + 2.0*pi/3.0);
				
                elseif (InjectMode == 2)
					ua = InjectAmp * sin(omega * clock_t);
					ub = InjectAmp * sin(omega * clock_t + 2.0*pi/3.0);
					uc = InjectAmp * sin(omega * clock_t - 2.0*pi/3.0);
                    
                elseif (InjectMode == 3)
                    ua = InjectAmp * sin(omega * clock_t);
					ub = 0.5 * InjectAmp * sin(omega * clock_t + 2.0*pi/3.0) + ...
                         0.5 * InjectAmp * sin(omega * clock_t - 2.0*pi/3.0);
					uc = ub;
                else
                    % other InjectMode to be write here.
                end
			else 
				ua = 0; ub = 0; uc = 0;
            end
			
		
        elseif (hFreqInScan > FreqEnd ) 
			status_code = 2;
			hFreqInScan = 0;
			ua = 0; ub = 0; uc = 0;
		
		else 
			status_code = 3;
        end

    else
		if (hStartFlagMem == 0)
			hFreqInScan = FreqBegin;
			status_code = -1;
        else
			status_code = 0;
			disturb_flag = 0;
			rec_flag = 0;
			rest_flag = 0;
			hStepCounter = int32(0);
			clock_t = double(hStepCounter) * SAMPLE_TIME;
			ua = 0; ub = 0; uc = 0;
        end
    end


	hStartFlagMem = int32(start_flag);  % record start_flag
	OutUa = ua;
	OutUb = ub;
	OutUc = uc;

	OutStatus = status_code;
	OutFreqInScan = hFreqInScan;
	OutClock = clock_t;
	OutDisturbFlag = disturb_flag;
	OutRecFlag = rec_flag;
	OutRestFlag = rest_flag;
    OutPosOrNegFlag = InjectMode;
end
